simulink model "multiRobotSoccer"  (R2026b)
settings: Solver=FixedStepAuto  StopTime=inf  FixedStep=sampleTime
PreLoadFcn:
  | robotSoccerParams;
values from neighbouring files (symbols this model uses):
  angThresh = pi/16    (= 0.196349540849)    [robotSoccerParams.m]
  attackerKickSpeed = 3    [robotSoccerParams.m]
  attackerMaxGoalDist = 10    [robotSoccerParams.m]
  attackerMinGoalDist = 5    [robotSoccerParams.m]
  awayGoalPosition = [fieldLimitsX(2) mean(fieldLimitsY)]    [robotSoccerParams.m]
  ballAngleNoise = pi/24    (= 0.1308996939)    [robotSoccerParams.m]
  ballThresh = robotRadius + 0.3    (= 1.1)    [robotSoccerParams.m]
  ballVelNoise = 0.5    [robotSoccerParams.m]
  defenderAwayPoses = [72 28.5 pi ... (first row only)    [robotSoccerParams.m]
  defenderHomePoses = [20 28.5 0 ... (first row only)    [robotSoccerParams.m]
  defenderKickSpeed = 5    [robotSoccerParams.m]
  distThresh = 1    [robotSoccerParams.m]
  dribbleKickSpeed = 2    [robotSoccerParams.m]
  dribbleTime = 25    [robotSoccerParams.m]
  fieldCenter = [mean(fieldLimitsX) mean(fieldLimitsY)]    [robotSoccerParams.m]
  fieldLimitsX = [0 92]    [robotSoccerParams.m]
  fieldLimitsY = [0 47]    [robotSoccerParams.m]
  goalkeeperKickSpeed = 10    [robotSoccerParams.m]
  goalkeeperPoses = [ 2 23.5 0 ... (first row only)    [robotSoccerParams.m]
  goalPosts = [ 0 27.15 2 ... (first row only)    [robotSoccerParams.m]
  goalThresh = 20    [robotSoccerParams.m]
  homeGoalPosition = [fieldLimitsX(1) mean(fieldLimitsY)]    [robotSoccerParams.m]
  initBallPos = fieldCenter    [robotSoccerParams.m]
  initGameState = struct('possession',0,                         'state',GameState.InPlay,                         'score',[0;0])    [robotSoccerParams.m]
  numRobots = 6    [robotSoccerParams.m]
  outOfBoundsDist = 2    [robotSoccerParams.m]
  robotDetectorMaxHits = 5    [robotSoccerParams.m]
  robotRadius = 0.8    [robotSoccerParams.m]
undefined symbols (not defined in the file or in its folder): DiscIntNeverNeededParam, ObjectType
libraries: soccerRobotLib x6, mobileRoboticsLib x1
settings Model: TunableVars=angThresh,attackerKickSpeed,attackerMaxGoalDist,attackerMinGoalDist,awayGoalPosition,ballAngleNoise,ballCarryFactor,ballThresh,ballVelNoise,defenderAwayPoses,defenderHomePoses,defenderKickSpeed,distThresh,dribbleKickSpeed,dribbleTime,fieldCenter,fieldLimitsX,fieldLimitsY,goalPosts,goalThresh,goalkeeperKickSpeed,goalkeeperPoses,homeGoalPosition,initBallPos,initGameState,initialPoses,numRobots,objColors,objDetectorAngle,objDetectorFOV,objDetectorMaxHits,objDetectorOffset,objDetectorRange,outOfBoundsDist,robotColors,robotDetectorAngle,robotDetectorFOV,robotDetectorMaxHits,robotDetectorOffset,robotDetectorRange,robotRadius,sampleTime,wheelRadius  TunableVarsStorageClass=Auto,Auto,Auto,Auto,Auto,Auto,Auto,Auto,Auto,Auto,Auto,Auto,Auto,Auto,Auto,Auto,Auto,Auto,Auto,Auto,Auto,Auto,Auto,Auto,Auto,Auto,Auto,Auto,Auto,Auto,Auto,Auto,Auto,Auto,Auto,Auto,Auto,Auto,Auto,Auto,Auto,Auto,Auto  TunableVarsTypeQualifier=,,,,,,,,,,,,,,,,,,,,,,,,,,,,,,,,,,,,,,,,,,  Creator=scastro  LastModifiedBy=fayne
settings DataIOCC: ReturnWorkspaceOutputs=off
settings OptimizationCC: DifferentSizesBufferReuse=on  EfficientTunableParamExpr=on  EnhancedBackFolding=on  OptimizationCustomize=off  OptimizeBlockOrder=speed  PassReuseOutputArgsAs=Individual arguments
settings DebuggingCC: ArithmeticOperatorsInVariantConditions=warning  BusObjectLabelMismatch=error  NonBusSignalsTreatedAsBus=error  ParameterTunabilityLossMsg=error  StrictBusMsg=ErrorOnBusTreatedAsVector
settings SFSimCC: CustomCodeUndefinedFunction=UseInterfaceOnly  MATLABDynamicMemAlloc=off  SimUseLocalCustomCode=off
settings RTWCC: Description=Embedded Coder  GenerateReport=on  GenerateTraceInfo=on  GenerateTraceReport=on  GenerateTraceReportEml=on  GenerateTraceReportSf=on  GenerateTraceReportSl=on  GenerateWebview=on  IncludeHyperlinkInReport=on  LaunchReport=on  RTWUseLocalCustomCode=off  SystemTargetFile=ert.tlc  TemplateMakefile=ert_default_tmf
settings CodeAppCC: ForceParamTrailComments=on  IgnoreCustomStorageClasses=off  InsertBlockDesc=on  OperatorAnnotations=on  SFDataObjDesc=on  SimulinkDataObjDesc=on
settings ERTTargetCC: DynamicArrayContainerType=coder::array  GenerateSampleERTMain=on  SupportVariableSizeSignals=on

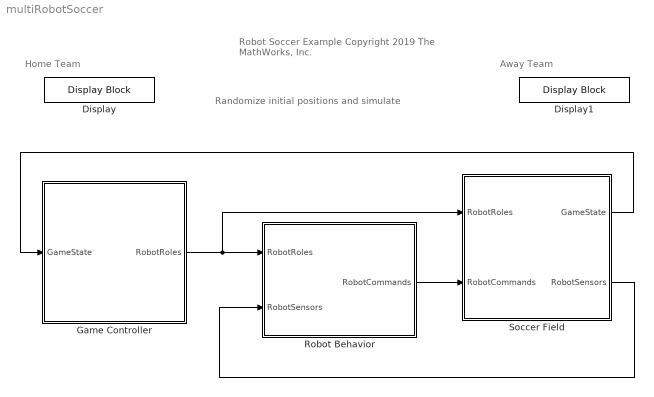
== system multiRobotSoccer ==
  note: Home Team
  note: Randomize initial positions and simulate
  note: Robot Soccer Example
      | Copyright 2019 The MathWorks, Inc.
  note: Away Team
  Display : DisplayBlock  LabelPosition=Hide  Format=long  GridColor=[0.502, 0.502, 0.502]
  Display1 : DisplayBlock  LabelPosition=Hide  Format=long  GridColor=[0.502, 0.502, 0.502]
  Game Controller : Subsystem
  Robot Behavior : Subsystem
  Soccer Field : Subsystem
  wires:
  Robot Behavior/1(RobotCommands) -> Soccer Field/2(RobotCommands)
  Game Controller/1(RobotRoles) -> Soccer Field/1(RobotRoles), Robot Behavior/1(RobotRoles)
  Soccer Field/1(GameState) -> Game Controller/1(GameState)
  Soccer Field/2(RobotSensors) -> Robot Behavior/2(RobotSensors)

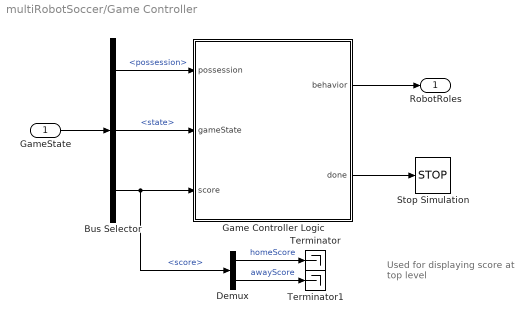
== system multiRobotSoccer/Game Controller ==
  note: Used for displaying score at top level
  GameState : Inport
  Bus Selector : BusSelector  OutputSignals=possession,state,score
  Demux : Demux  Outputs=2
  Game Controller Logic : Stateflow chart  TreatAsAtomicUnit=on
  Stop Simulation : Stop
  Terminator : Terminator
  Terminator1 : Terminator
  RobotRoles : Outport  VectorParamsAs1DForOutWhenUnconnected=off
  wires:
  Game Controller Logic/1(behavior) -> RobotRoles/1
  GameState/1 -> Bus Selector/1
  Bus Selector/1 -> Game Controller Logic/1(possession)  "<possession>"
  Bus Selector/2 -> Game Controller Logic/2(gameState)  "<state>"
  Bus Selector/3 -> Demux/1, Game Controller Logic/3(score)  "<score>"
  Demux/1 -> Terminator/1  "homeScore"
  Demux/2 -> Terminator1/1  "awayScore"
  Game Controller Logic/2(done) -> Stop Simulation/1

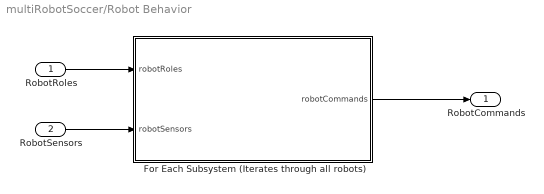
== system multiRobotSoccer/Robot Behavior ==
  RobotRoles : Inport
  RobotSensors : Inport  Port=2
  For Each Subsystem (Iterates through all robots) : Subsystem  TreatAsAtomicUnit=on
  RobotCommands : Outport  OutDataTypeStr=Bus: RobotCommandBus  PortDimensions=2  VectorParamsAs1DForOutWhenUnconnected=off
  wires:
  RobotRoles/1 -> For Each Subsystem (Iterates through all robots)/1(robotRoles)
  RobotSensors/1 -> For Each Subsystem (Iterates through all robots)/2(robotSensors)
  For Each Subsystem (Iterates through all robots)/1(robotCommands) -> RobotCommands/1

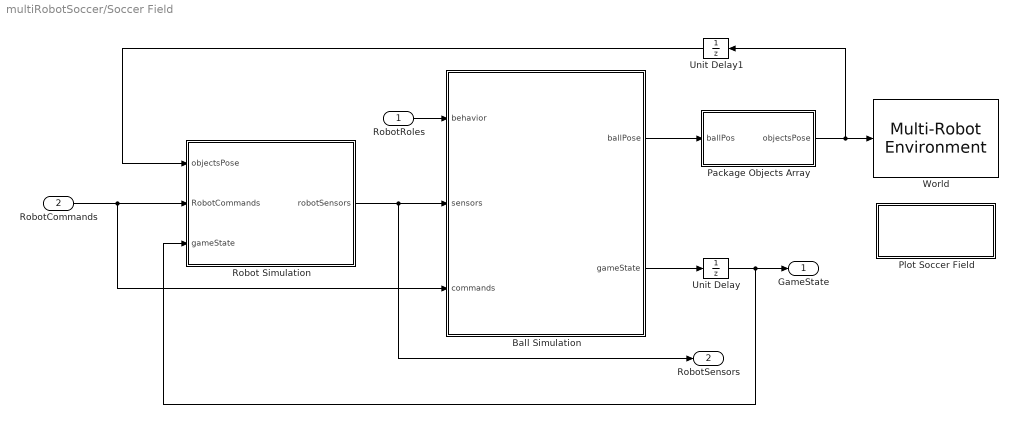
== system multiRobotSoccer/Soccer Field ==
  RobotRoles : Inport
  RobotCommands : Inport  Port=2
  Ball Simulation : Stateflow chart  TreatAsAtomicUnit=on
  Package Objects Array : Subsystem
  Plot Soccer Field : MATLAB Function  TreatAsAtomicUnit=on
  Robot Simulation : Subsystem
  Unit Delay : UnitDelay  InitialCondition=initGameState  SampleTime=-1
  Unit Delay1 : UnitDelay  InitialCondition=[initBallPos double(ObjectType.Ball); goalPosts]  SampleTime=-1
  World : mobileRoboticsLib/Environments/Multi-Robot Environment  numRobots=numRobots  mapName=map  showWaypoints=off  showObjects=on  objectColors=objColors  objectMarkers=objMarkers  showRobotIds=off  plotSensorLines=off
      settings: SourceProductName=Mobile Robotics Simulation Toolbox
  GameState : Outport  VectorParamsAs1DForOutWhenUnconnected=off
  RobotSensors : Outport  Port=2  VectorParamsAs1DForOutWhenUnconnected=off
  wires:
  Package Objects Array/1(objectsPose) -> World/1, Unit Delay1/1
  Ball Simulation/1(ballPose) -> Package Objects Array/1(ballPos)
  RobotCommands/1 -> Robot Simulation/2(RobotCommands), Ball Simulation/3(commands)
  Ball Simulation/2(gameState) -> Unit Delay/1
  Unit Delay1/1 -> Robot Simulation/1(objectsPose)
  Unit Delay/1 -> Robot Simulation/3(gameState), GameState/1
  Robot Simulation/1(robotSensors) -> RobotSensors/1, Ball Simulation/2(sensors)
  RobotRoles/1 -> Ball Simulation/1(behavior)

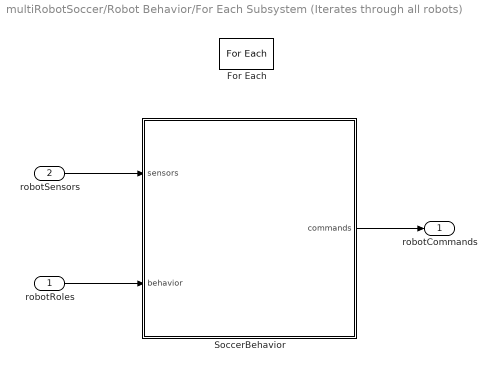
== system multiRobotSoccer/Robot Behavior/For Each Subsystem (Iterates through all robots) ==
  robotRoles : Inport  Partition=on  PartitionDimension=1  PartitionWidth=1  PartitionOffset=0
  robotSensors : Inport  Port=2  Partition=on  PartitionDimension=1  PartitionWidth=1  PartitionOffset=0
  For Each : ForEach  DisableCoverage=on
  SoccerBehavior : Stateflow chart  TreatAsAtomicUnit=on
  robotCommands : Outport  ConcatenationDimension=1  VectorParamsAs1DForOutWhenUnconnected=off
  wires:
  SoccerBehavior/1(commands) -> robotCommands/1
  robotRoles/1 -> SoccerBehavior/2(behavior)
  robotSensors/1 -> SoccerBehavior/1(sensors)

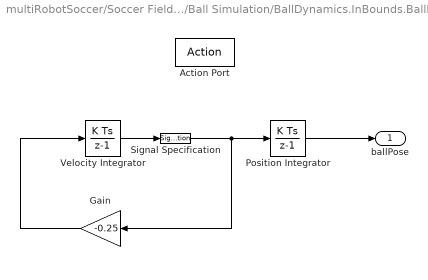
== system multiRobotSoccer/Soccer Field/Ball Simulation/BallDynamics.InBounds.BallFree ==
  Action Port : ActionPort
      settings: CopyFcn=Stateflow.SLINSF.SimulinkMan.removeBlockPreDeleteFcn  PreDeleteFcn=Stateflow.SLINSF.SimulinkMan.unsafePredeleteFcn
  Gain : Gain  Gain=-0.25
  Position Integrator : DiscreteIntegrator  InitialCondition=initBallPos  SampleTime=-1  StateName=ballPos  ICPrevOutput=DiscIntNeverNeededParam  ICPrevScaledInput=DiscIntNeverNeededParam
  Signal Specification : SignalSpecification  Dimensions=[1 2]
  Velocity Integrator : DiscreteIntegrator  InitialCondition=[0 0]  SampleTime=-1  StateName=ballVel  ICPrevOutput=DiscIntNeverNeededParam  ICPrevScaledInput=DiscIntNeverNeededParam
  ballPose : Outport  VectorParamsAs1DForOutWhenUnconnected=off
  wires:
  Gain/1 -> Velocity Integrator/1
  Velocity Integrator/1 -> Signal Specification/1
  Position Integrator/1 -> ballPose/1
  Signal Specification/1 -> Position Integrator/1, Gain/1

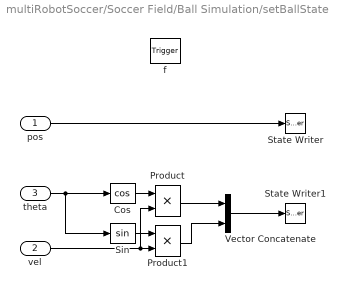
== system multiRobotSoccer/Soccer Field/Ball Simulation/setBallState ==
  pos : Inport  OutDataTypeStr=double  PortDimensions=[1 2]
  vel : Inport  Port=2  OutDataTypeStr=double  PortDimensions=1
  theta : Inport  Port=3  OutDataTypeStr=double  PortDimensions=1
  f : TriggerPort  TriggerType=function-call  VariantControl=(inherit)
      settings: CopyFcn=Stateflow.SLINSF.SimulinkMan.removeBlockPreDeleteFcn  PreDeleteFcn=Stateflow.SLINSF.SimulinkMan.unsafePredeleteFcn
  Cos : Trigonometry  Operator=cos
  Product : Product
  Product1 : Product
  Sin : Trigonometry
  State Writer : StateWriter  StateOwnerBlock=../../BallDynamics.InBounds.BallFree/Position Integrator  StateName=ballPos
  State Writer1 : StateWriter  StateOwnerBlock=../../BallDynamics.InBounds.BallFree/Velocity Integrator  StateName=ballVel
  Vector Concatenate : Concatenate  Mode=Multidimensional array  ConcatenateDimension=2
  wires:
  Vector Concatenate/1 -> State Writer1/1
  Product1/1 -> Vector Concatenate/2
  Product/1 -> Vector Concatenate/1
  theta/1 -> Cos/1, Sin/1
  Sin/1 -> Product1/1
  vel/1 -> Product1/2, Product/2
  Cos/1 -> Product/1
  pos/1 -> State Writer/1

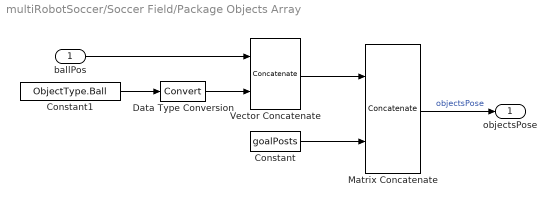
== system multiRobotSoccer/Soccer Field/Package Objects Array ==
  ballPos : Inport
  Constant : Constant  Value=goalPosts  VectorParams1D=off
  Constant1 : Constant  Value=ObjectType.Ball
  Data Type Conversion : DataTypeConversion  SaturateOnIntegerOverflow=off  RndMeth=Floor
  Matrix Concatenate : Concatenate  Mode=Multidimensional array
  Vector Concatenate : Concatenate  Mode=Multidimensional array  ConcatenateDimension=2
  objectsPose : Outport  VectorParamsAs1DForOutWhenUnconnected=off
  wires:
  Constant/1 -> Matrix Concatenate/2
  Matrix Concatenate/1 -> objectsPose/1  "objectsPose"
  Vector Concatenate/1 -> Matrix Concatenate/1
  ballPos/1 -> Vector Concatenate/1
  Constant1/1 -> Data Type Conversion/1
  Data Type Conversion/1 -> Vector Concatenate/2

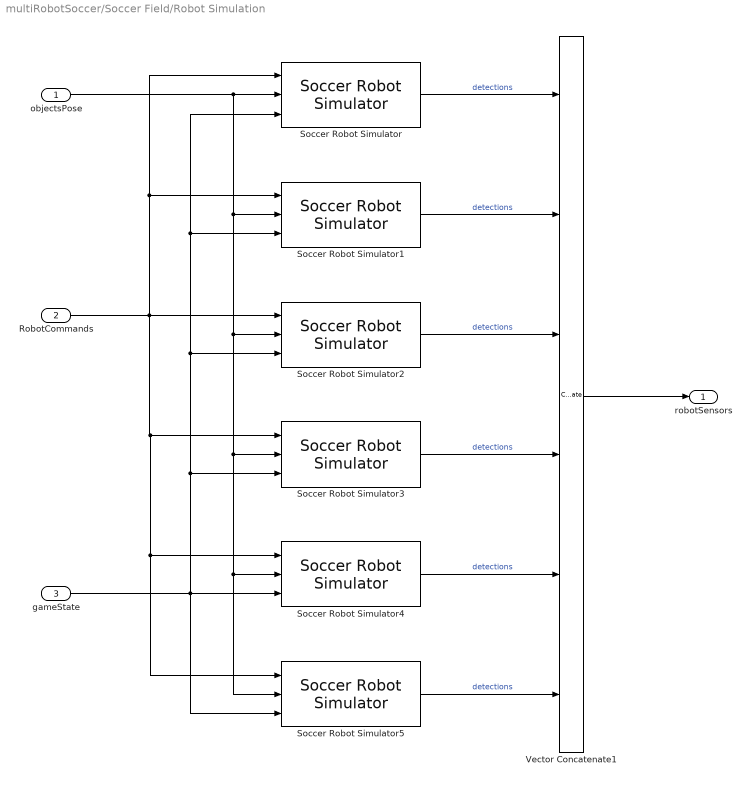
== system multiRobotSoccer/Soccer Field/Robot Simulation ==
  objectsPose : Inport
  RobotCommands : Inport  Port=2
  gameState : Inport  Port=3
  Soccer Robot Simulator : soccerRobotLib/Soccer Robot Simulator  robotIdx=1
  Soccer Robot Simulator1 : soccerRobotLib/Soccer Robot Simulator  robotIdx=2
  Soccer Robot Simulator2 : soccerRobotLib/Soccer Robot Simulator  robotIdx=3
  Soccer Robot Simulator3 : soccerRobotLib/Soccer Robot Simulator  robotIdx=4
  Soccer Robot Simulator4 : soccerRobotLib/Soccer Robot Simulator  robotIdx=5
  Soccer Robot Simulator5 : soccerRobotLib/Soccer Robot Simulator  robotIdx=6
  Vector Concatenate1 : Concatenate  NumInputs=6
  robotSensors : Outport  VectorParamsAs1DForOutWhenUnconnected=off
  wires:
  RobotCommands/1 -> Soccer Robot Simulator/1, Soccer Robot Simulator1/1, Soccer Robot Simulator5/1, Soccer Robot Simulator4/1, Soccer Robot Simulator3/1, Soccer Robot Simulator2/1
  objectsPose/1 -> Soccer Robot Simulator/2, Soccer Robot Simulator1/2, Soccer Robot Simulator5/2, Soccer Robot Simulator4/2, Soccer Robot Simulator3/2, Soccer Robot Simulator2/2
  Vector Concatenate1/1 -> robotSensors/1
  Soccer Robot Simulator/1 -> Vector Concatenate1/1  "detections"
  Soccer Robot Simulator1/1 -> Vector Concatenate1/2  "detections"
  Soccer Robot Simulator2/1 -> Vector Concatenate1/3  "detections"
  Soccer Robot Simulator3/1 -> Vector Concatenate1/4  "detections"
  gameState/1 -> Soccer Robot Simulator5/3, Soccer Robot Simulator/3, Soccer Robot Simulator1/3, Soccer Robot Simulator2/3, Soccer Robot Simulator3/3, Soccer Robot Simulator4/3
  Soccer Robot Simulator4/1 -> Vector Concatenate1/5  "detections"
  Soccer Robot Simulator5/1 -> Vector Concatenate1/6  "detections"

== stateflow chart multiRobotSoccer/Soccer Field/Ball Simulation ==
  state BallPossession [parallel]
    en:
    gameState.possession = 0;
    en,du:
    % Calculate distances from robots to ball
    % (Goalkeepers get 2x the range)
    for idx = 1:numRobots
    ballDists(idx) = norm( sensors(idx).pose(1:2) - ballPose' );
    if behavior(idx).role == Role.Goalkeeper
    ballDists(idx) = ballDists(idx)/2;
    end
    end
    % Find the robot index of the current and latest possessions
    robotIdx = findPossession;
    if robotIdx > 0
    lastPossession = robotIdx;
    end
    % Unpack the robot commands
    action = commands(lastPossession).action;
    ballVel = commands(lastPossession).ballVelocity;
    robotPose = sensors(lastPossession).pose;
    settings: executionOrder=1
  state BallDynamics [parallel]
    en:
    coder.extrinsic('randn'); % Lets us use MATLAB's interpreted RNG
    setBallState(initBallPos,0,0);
    settings: executionOrder=2
    state InBounds
      en, du:
      randNum = randn(2,1);
      gameState.state = getGameState;
      state BallFree
      state BallHeld
        en: gameState.possession = robotIdx;
        en,du:
        ballPose = [robotPose(1) robotPose(2)] + ...
        (robotRadius+ballThresh)*[cos(robotPose(3)) sin(robotPose(3))];
      (default) -> BallFree
      BallHeld -> BallFree : [action == RobotAction.KickBall]
          | {setBallState(ballPose,ballVel + ballVelNoise*randNum(1), ...
          |  robotPose(3) + ballAngleNoise*randNum(2));
          | gameState.possession = 0;}
      BallFree -> BallHeld : [after(2,sec) && ...
          |  robotIdx > 0]
    state OutOfBounds
      en:
      % If a goal is scored, increment the score
      if gameState.state == GameState.GoalScored
      ballPose = initBallPos;
      teamIdx = behavior(lastPossession).team;
      gameState.score(teamIdx) = gameState.score(teamIdx) + 1;
      % Else, place the ball back in bounds
      else
      ballPose = placeBallInBounds();
      end
      setBallState(ballPose,0,robotPose(3));
    (default) -> InBounds
    OutOfBounds -> InBounds : after(1,sec)
    InBounds -> OutOfBounds : [gameState.state ~= GameState.InPlay]
  state setBallState(pos,vel,theta) [function]
  state rIdx = findPossession [function]
    (default) -> (junction 125)
    (junction 125) -> (junction 127) [order 1] : % If the robot that previously possessed the ball is still holding it, keep the same index
        | [(gameState.possession > 0) && ...
        | (commands(gameState.possession).action == RobotAction.HoldBall)]
    (junction 125) -> (junction 131) [order 2] : % Else, find another valid robot holder
        | {rIdx = findNearestHoldingRobot;}
    (junction 127) -> (junction 129) : {rIdx = gameState.possession;}
    (junction 129) -> (junction 131)
  state state = getGameState [function]
    note: Returns the game state depending on the position of the ball on the field
    (default) -> (junction 98)
    (junction 98) -> (junction 100) [order 1] : [ballPose(1) <= fieldLimitsX(1) || ballPose(1) >= fieldLimitsX(2) || ...
        |  ballPose(2) <= fieldLimitsY(1) || ballPose(2) >= fieldLimitsY(2)]
    (junction 98) -> (junction 111) [order 2] : {state = GameState.InPlay;}
    (junction 100) -> (junction 102)
    (junction 102) -> (junction 104) [order 1] : [ballPose(2)<=goalPosts(1,2) && ...
        | ballPose(2) >= goalPosts(2,2)]
    (junction 102) -> (junction 108) [order 2] : {state = GameState.OutOfPlay;}
    (junction 104) -> (junction 106) : {state = GameState.GoalScored;}
    (junction 108) -> (junction 111)
    (junction 106) -> (junction 108)
  state newPose = placeBallInBounds [function]
    note: Calculates the new pose of the ball when returning from out of bounds
    (default) -> (junction 90) : {
        | newPose = [ ...
        |  max( fieldLimitsX(1)+outOfBoundsDist , min(ballPose(1),fieldLimitsX(2)-outOfBoundsDist) ), ...
        | max( fieldLimitsY(1)+outOfBoundsDist , min(ballPose(2),fieldLimitsY(2)-outOfBoundsDist) ) ...
        | ];
        | }
  data: sf_internal_action_state_placeholder_data local double size=1 =0; pos function_input double size=[1 2]; vel function_input double size=1; theta function_input double size=1; nearIdx function_output size=1; rIdx function_output; state function_output; newPose function_output; behavior input Bus: RobotBehaviorBus; sensors input Bus: RobotSensorBus size=numRobots; ballPose output; commands input Bus: RobotCommandBus size=numRobots; robotRadius parameter; robotPose local =[0 0 0]'; action local =RobotAction.DoNothing; gameState output Bus: GameStateBus size=1; robotIdx local =1; lastPossession local =1; initBallPos parameter; randNum local =[0;0]; teamIdx local =1; ballVel local =0; ballThresh parameter; numRobots parameter; idx local =0; ballVelNoise parameter; ballAngleNoise parameter; outOfBoundsDist parameter; fieldLimitsY parameter; fieldLimitsX parameter; ballDists local =zeros(numRobots,1); goalPosts parameter
  function nearIdx = findNearestHoldingRobot:
    | function rIdx = findNearestHoldingRobot
    | % Finds possession based on the commands to all the robots 
    | % and their distances to the ball
    | 
    | [~,inds] = sort(ballDists);
    | rIdx = 0;
    | for idx = 1:numRobots
    |     if (commands(inds(idx)).action == RobotAction.HoldBall) && ....
    |        (ballDists(inds(idx)) <= ballThresh)
    |         rIdx = inds(idx);
    |         return;
    |     end
    | end
    | 
    | end

== matlab function multiRobotSoccer/Soccer Field/Plot Soccer Field ==
function plotSoccerField
% Plots the soccer field once the figure window for the environment has
% been initialized

coder.extrinsic('evalin');
persistent hasPlotted
if isempty(hasPlotted)
    evalin('base','plotSoccerField');
    hasPlotted = true;
end

== stateflow chart multiRobotSoccer/Game Controller/Game Controller Logic ==
  state GameOn
    en:
    done = false;
    % Assign player strategy
    assignRobotStrategies
    % Constantly check possession
    en,du:
    if possession > 0
    posTeam = behavior(possession).team;
    else
    posTeam = 0;
    end
    for idx = 1:numRobots
    behavior(idx).possessingTeam = posTeam;
    end
    state HomeTeamAttacks
      en:
      behavior(1).role = Role.Goalkeeper;
      behavior(2).role = Role.Goalkeeper;
      behavior(3).role = Role.Attacker;
      behavior(4).role = Role.Defender;
      behavior(5).role = Role.Attacker;
      behavior(6).role = Role.Defender;
    state HomeTeamDefends
      en:
      behavior(1).role = Role.Goalkeeper;
      behavior(2).role = Role.Goalkeeper;
      behavior(3).role = Role.Defender;
      behavior(4).role = Role.Attacker;
      behavior(5).role = Role.Defender;
      behavior(6).role = Role.Attacker;
    (default) -> HomeTeamAttacks
    HomeTeamAttacks -> HomeTeamDefends : [hasChangedFrom(gameState,GameState.InPlay) || ...
        |  posTeam == 2]
    HomeTeamDefends -> HomeTeamAttacks : [hasChangedFrom(gameState,GameState.InPlay) || ...
        |  posTeam == 1]
  state assignRobotStrategies [function]
    note: Assigns initial robot teams, roles, and default formation poses
    (default) -> (junction 54) : {
        | % Assign teams
        | behavior(1).team = 1;
        | behavior(2).team = 2;
        | behavior(3).team = 1;
        | behavior(4).team = 2;
        | behavior(5).team = 1;
        | behavior(6).team = 2;
        | }
    (junction 54) -> (junction 56) : {
        | % Assign goalkeeper roles and default poses
        | behavior(1).role = Role.Goalkeeper;
        | behavior(1).formationPose = goalkeeperPoses(:,1);
        | behavior(2).role = Role.Goalkeeper;
        | behavior(2).formationPose = goalkeeperPoses(:,2);
        | }
    (junction 56) -> (junction 58) : {
        | % Assign defender default poses
        | behavior(3).formationPose = defenderHomePoses(:,1);
        | behavior(4).formationPose = defenderAwayPoses(:,1);
        | behavior(5).formationPose = defenderHomePoses(:,2);
        | behavior(6).formationPose = defenderAwayPoses(:,2);
        | }
  state GameOver
    en:
    done = true;
  (default) -> GameOn
  GameOn -> GameOver : % End the game when a team scores 5
      | [any(score >= 5)]
  data: possession input; gameState input; score input; behavior output Bus: RobotBehaviorBus size=numRobots; numRobots local =numRobots; idx local =1; posTeam local size=1 =0; defenderAwayPoses parameter; defenderHomePoses parameter; goalkeeperPoses parameter; done output

== stateflow chart multiRobotSoccer/Robot Behavior/For Each Subsystem (Iterates through all robots)/SoccerBehavior ==
  settings: updateMethod=DISCRETE  sampleTime=sampleTime
  state ExecuteBehavior [parallel]
    en,du:
    prevRole = behavior.role;
    settings: executionOrder=1
    state Attack
      % Attack logic: Go to the ball, carry it near the goal, and shoot!
      en:
      if behavior.team == 1
      goalPose = [awayGoalPosition';0];
      else
      goalPose = [homeGoalPosition';pi];
      end
      state GoToBall
        en:
        commands.action = RobotAction.HoldBall;
        en,du:
        [ballRange,ballAngle] = detectBall(sensors.detections);
        commands.robotVelocity = trackDetection(ballRange,ballAngle);
      state KickBall
        en:
        commands.action = RobotAction.KickBall;
        commands.robotVelocity = [0;0;0];
        commands.ballVelocity = attackerKickSpeed;
      state GoToGoal
        en:
        commands.action = RobotAction.HoldBall;
        en,du:
        [goalDistance,goalAngle] = calcBearing(goalPose);
        commands.robotVelocity = goToPose(goalPose);
      state Dribble
        %Dribble the ball if held for too long
        en:
        commands.action = RobotAction.KickBall;
        commands.ballVelocity = dribbleKickSpeed;
      state BackUp
        % Move out of goal if too close
        en:
        commands.action = RobotAction.HoldBall;
        en,du:
        commands.robotVelocity = goToPose([fieldCenter';pi/2]);
      (default) -> GoToBall
      GoToBall -> ExecuteBehavior.Attack.GoToGoal : [sensors.ballHeld]
      ExecuteBehavior.Attack.KickBall -> GoToBall : [after(1,sec)]
      ExecuteBehavior.Attack.GoToGoal -> ExecuteBehavior.Attack.KickBall [order 2] : [goalDistance <= goalThresh && ...
          |  abs(goalAngle) < angThresh]
      ExecuteBehavior.Attack.GoToGoal -> Dribble [order 3] : [after(dribbleTime,sec)]
      Dribble -> ExecuteBehavior.Attack.GoToGoal : [after(0.5,sec)]
      ExecuteBehavior.Attack.GoToGoal -> BackUp [order 1] : [abs(sensors.pose(1) - goalPose(1)) < ...
          | attackerMinGoalDist]
      BackUp -> ExecuteBehavior.Attack.GoToGoal : [abs(sensors.pose(1) - goalPose(1)) > ...
          | attackerMaxGoalDist]
    state Defend
      % Defense logic: If own team has ball possession, go to the goal. Else, chase after the ball.
      state DefensiveActions
        en,du:
        ballRange = detectBall(sensors.detections);
        state DefendGoal
          en:
          commands.action = RobotAction.HoldBall;
          goalPose = behavior.formationPose;
          en,du:
          commands.robotVelocity = goToPose(goalPose);
        state ChaseBall
          en,du:
          if behavior.possessingTeam == 0
          commands.action = RobotAction.HoldBall;
          else
          commands.action = RobotAction.DoNothing;
          end
          [ballRange,ballAngle] = detectBall(sensors.detections);
          commands.robotVelocity = trackDetection(ballRange,ballAngle);
        (default) -> DefendGoal
        ChaseBall -> DefendGoal : [behavior.possessingTeam == behavior.team]
        DefendGoal -> ChaseBall : [behavior.possessingTeam == 0 ...
            |  && distToOwnGoal < diff(fieldLimitsX)/2 && ...
            |  ballRange < diff(fieldLimitsX)/2 && ballRange > 0]
      state TurnToGoal
        en:
        if behavior.team == 1
        goalPose = [awayGoalPosition';0];
        else
        goalPose = [homeGoalPosition';pi];
        end
        en,du:
        commands.action = RobotAction.HoldBall;
        [commands.robotVelocity,isdone] = turnToPoint(goalPose);
      state KickBall
        en:
        commands.action = RobotAction.KickBall;
        commands.robotVelocity = [0;0;0];
        commands.ballVelocity = defenderKickSpeed;
      state dist = distToOwnGoal [function]
        (default) -> (junction 441)
        (junction 441) -> (junction 444) [order 1] : [behavior.team == 1]
        (junction 441) -> (junction 448) [order 2] : {dist = calcBearing(awayGoalPosition');}
        (junction 444) -> (junction 446) : {dist = calcBearing(homeGoalPosition');}
        (junction 446) -> (junction 448)
      (default) -> DefensiveActions
      DefensiveActions -> TurnToGoal : [sensors.ballHeld]
      TurnToGoal -> ExecuteBehavior.Defend.KickBall : [isdone || after(10,sec)]
      ExecuteBehavior.Defend.KickBall -> DefensiveActions : [after(1,sec)]
    state Goalkeep
      % Goalkeeper logic: Wait for the ball and try hold it if nearby. If the ball is held, kick it far away!
      en:
      goalPose = behavior.formationPose;
      state GoalkeeperActions
        en, du:
        [ballRange,ballAngle] = detectBall(sensors.detections);
        state TurnToBall
          en:
          commands.robotVelocity = [0;0;0];
          commands.action = RobotAction.HoldBall;
          en,du:
          if ballAngle > angThresh
          commands.robotVelocity(3) = 1;
          elseif ballAngle < -angThresh
          commands.robotVelocity(3) = -1;
          else
          commands.robotVelocity(3) = 0;
          end
        state GoToGoal
          en,du:
          [commands.robotVelocity,isdone] = goToPose(goalPose);
          commands.action = RobotAction.HoldBall;
        (default) -> ExecuteBehavior.Goalkeep.GoalkeeperActions.GoToGoal
        ExecuteBehavior.Goalkeep.GoalkeeperActions.GoToGoal -> TurnToBall : [isdone && ballRange > 0]
        TurnToBall -> ExecuteBehavior.Goalkeep.GoalkeeperActions.GoToGoal : [ballRange < 0]
      state TurnToCenterline
        en,du:
        commands.robotVelocity = ...
        goToPose([fieldCenter';0]);
      state KickBall
        en:
        commands.robotVelocity = [0;0;0];
        commands.action = RobotAction.KickBall;
        commands.ballVelocity = goalkeeperKickSpeed;
      (default) -> GoalkeeperActions
      GoalkeeperActions -> TurnToCenterline : [sensors.ballHeld]
      ExecuteBehavior.Goalkeep.KickBall -> GoalkeeperActions : [after(1,sec)]
      TurnToCenterline -> ExecuteBehavior.Goalkeep.KickBall : [after(3,sec)]
    state DoNothing
      % Do not move, and do not do anything with the ball.
      en:
      commands.action = RobotAction.DoNothing;
      commands.robotVelocity = [0;0;0];
    (default) -> (junction 348)
    ExecuteBehavior -> (junction 348) : [behavior.role ~= prevRole]
    (junction 348) -> Attack [order 1] : [behavior.role==Role.Attacker]
    (junction 348) -> (junction 354) [order 2]
    Defend -> Attack : [behavior.possessingTeam == ...
        | behavior.team]
    Attack -> Defend : [behavior.possessingTeam == ...
        |  opposingTeam]
    (junction 354) -> Defend [order 1] : [behavior.role==Role.Defender]
    (junction 354) -> (junction 358) [order 2]
    (junction 358) -> Goalkeep [order 1] : [behavior.role==Role.Goalkeeper]
    (junction 358) -> (junction 361) [order 2]
    (junction 361) -> DoNothing
  state AvoidRobots [parallel]
    % All robots not holding the ball should avoid other robots using data from their Robot Detector sensors
    en,du:
    for idx = 1:robotDetectorMaxHits
    robotRanges(idx) = sensors.robotDetections(idx,1);
    end
    robotRanges(robotRanges<=0) = inf;
    [minRange,minRangeIdx] = min(robotRanges);
    settings: executionOrder=2
    state NormalOperation
      % Do not modify original commands to robot
    state Avoid
      en,du:
      % Move backwards and turn away from the commanded direction
      commands.robotVelocity(1) = -0.5;
      commands.robotVelocity(3) = -sign(sensors.robotDetections(minRangeIdx,2));
    (default) -> NormalOperation
    NormalOperation -> Avoid : [~sensors.ballHeld && ...
        | minRange < 3 && ~outOfBounds]
    Avoid -> NormalOperation : [after(1,sec) && ...
        | (~sensors.ballHeld || minRange > 5)]
  state [dist,ang] = calcBearing(goal) [function]
    (default) -> (junction 194) : % Calculate distance and angle to location
        | {
        | err = goal(1:2) - sensors.pose(1:2);
        | dist = norm(err);
        | ang = angdiff(sensors.pose(3),atan2(err(2),err(1)));
        | }
  state vel = trackDetection(dist,ang) [function]
    note: Uses range and bearing to track an object
    (default) -> (junction 321) : {
        | vel = [0;0;0];
        | }
    (junction 321) -> (junction 322) [order 1] : % Turn in place
        | % if no detection
        | [dist < 0]
    (junction 322) -> (junction 324) : {vel(3) = 1;}
    (junction 321) -> (junction 225) [order 2]
    (junction 225) -> (junction 229) [order 1] : % Forward speed
        | [dist > distThresh]
    (junction 225) -> (junction 231) [order 2]
    (junction 229) -> (junction 228) : {vel(1) = 1;}
    (junction 228) -> (junction 231)
    (junction 231) -> (junction 157)
    (junction 157) -> (junction 163) [order 1] : % Turning speed
        | [ang > angThresh]
    (junction 157) -> (junction 165) [order 2]
    (junction 163) -> (junction 172) : {vel(3) = 1;}
    (junction 165) -> (junction 167) [order 1] : [ang < -angThresh]
    (junction 165) -> (junction 162) [order 2]
    (junction 167) -> (junction 170) : {vel(3) = -1;}
    (junction 324) -> (junction 162)
    (junction 170) -> (junction 162)
    (junction 172) -> (junction 170)
  state [vel,done] = goToPose(goal) [function]
    note: Tracks a position. Once reached, the robot will turn in place until a reference angle is met.
    (default) -> (junction 247) : {
        | vel = [0;0;0];
        | [goalDist,goalAng] = calcBearing(goal(1:2));
        | trackAng = angdiff(sensors.pose(3),goal(3));
        | }
    (junction 247) -> (junction 248) [order 1] : % Track the position if outside the distance threshold
        | [goalDist > distThresh]
    (junction 247) -> (junction 299) [order 2] : % Else, turn in place until the angular reference is met
    (junction 248) -> (junction 280) : {vel = trackDetection(goalDist,goalAng);}
    (junction 299) -> (junction 300) [order 1] : [trackAng > angThresh]
    (junction 299) -> (junction 303) [order 2]
    (junction 300) -> (junction 284) : {vel(3) = 1;}
    (junction 303) -> (junction 305) [order 1] : [trackAng < -angThresh]
    (junction 303) -> (junction 310) [order 2]
    (junction 305) -> (junction 307) : {vel(3) = -1;}
    (junction 307) -> (junction 310)
    (junction 284) -> (junction 307)
    (junction 280) -> (junction 284)
    (junction 310) -> (junction 410) : {done = (goalDist <= distThresh) && (abs(trackAng) <= angThresh);}
  state [vel,done] = turnToPoint(goal) [function]
    note: Tracks a position. Once reached, the robot will turn in place until a reference angle is met.
    (default) -> (junction 375) : % Turn in place until the angular reference is met
        | {
        | done = false;
        | vel = [0;0;0];
        | [goalDist,goalAng] = calcBearing(goal(1:2));
        | }
    (junction 375) -> (junction 376) [order 1] : [goalAng > angThresh]
    (junction 375) -> (junction 377) [order 2]
    (junction 376) -> (junction 381) : {vel(3) = 1;}
    (junction 377) -> (junction 378) [order 1] : [goalAng < -angThresh]
    (junction 377) -> (junction 379) [order 2] : {done = true;}
    (junction 378) -> (junction 380) : {vel(3) = -1;}
    (junction 380) -> (junction 379)
    (junction 381) -> (junction 380)
  state flag = outOfBounds [function]
    note: Check whether a robot is out of bounds given a specified tolerance.
    (default) -> (junction 462) : {
        | flag = sensors.pose(1) <= fieldLimitsX(1)+outOfBoundsDist || ...
        |           sensors.pose(1) >= fieldLimitsX(2)-outOfBoundsDist || ...
        |           sensors.pose(2) <= fieldLimitsY(1)+outOfBoundsDist || ...
        |           sensors.pose(2) >= fieldLimitsY(2)-outOfBoundsDist;
        | }
  state team = opposingTeam [function]
    note: Convenience function that returns the number of the opposing team of a specific robot.
    (default) -> (junction 506)
    (junction 506) -> (junction 507) [order 1] : [behavior.team == 1]
    (junction 507) -> (junction 509) : {team = 2;}
    (junction 506) -> (junction 508) [order 2] : {team = 1;}
    (junction 509) -> (junction 508)
  data: dist function_output; goal function_input; dist function_output; ang function_output; dist function_input; ang function_input; vel function_output; vel function_output; done function_output; goal function_input; goal function_input; vel function_output; done function_output; flag function_output; team function_output; sensors input Bus: RobotSensorBus; behavior input; commands output Bus: RobotCommandBus; ballAngle local; ballRange local; goalPose local; distThresh parameter; goalThresh parameter; angThresh parameter; idx local =1; prevRole local =Role.None; isdone local =false; goalDistance local =0; goalAngle local =0; robotDetectorMaxHits parameter; homeGoalPosition parameter; awayGoalPosition parameter; fieldLimitsX parameter; fieldCenter parameter; fieldLimitsY parameter; minRangeIdx local; minRange local; robotRanges local =zeros(robotDetectorMaxHits,1); goalkeeperKickSpeed parameter; defenderKickSpeed parameter; attackerKickSpeed parameter; attackerMinGoalDist parameter; attackerMaxGoalDist parameter; dribbleKickSpeed parameter; dribbleTime parameter; outOfBoundsDist parameter double
